simulink model "Exp3_1"  (R2025b)
settings: Solver=VariableStepAuto  StartTime=0.0  StopTime=10.0  RelTol=1e-3
settings Model: Creator=SUBHASH  LastModifiedBy=SUBHASH
settings OptimizationCC: UseRowMajorAlgorithm=on

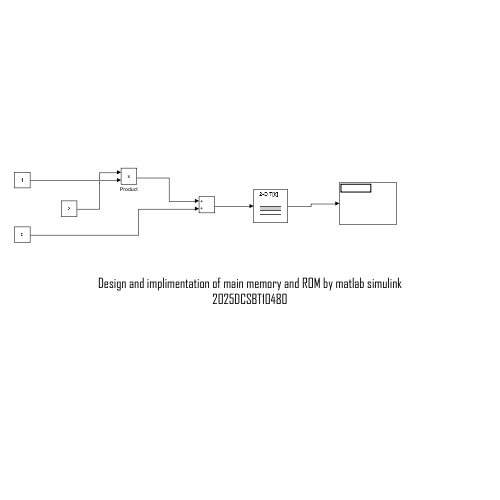
[thumbnail: Simulink's stored preview of the top-level diagram]
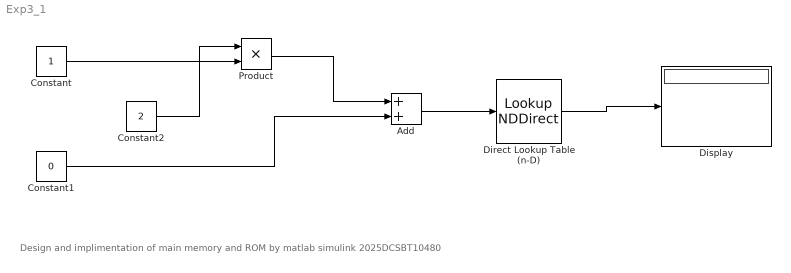
== system Exp3_1 ==
  note: Design and implimentation of main memory and ROM by matlab simulink
      | 2025DCSBT10480
  Add : Sum
  Constant : Constant
  Constant1 : Constant  Value=0
  Constant2 : Constant  Value=2
  Direct Lookup Table (n-D) : LookupNDDirect  InputsSelectThisObjectFromTable=Vector  Table=[1 0 0 0; 1 0 0 1; 1 0 1 0; 1 0 1 1]
  Display : Display
  Product : Product
  wires:
  Constant1/1 -> Add/2
  Constant/1 -> Product/2
  Product/1 -> Add/1
  Direct Lookup Table (n-D)/1 -> Display/1
  Add/1 -> Direct Lookup Table (n-D)/1
  Constant2/1 -> Product/1
